simulink model "mars_rover_terrain"  (R2025a)
settings: Solver=daessc  StartTime=0.0  StopTime=130*10  FixedStep=1e-10  MaxStep=1e-1  RelTol=1e-3  AbsTol=1e-3  EnableMultiTasking=on
undefined symbols (not defined in the file): arm_q0, Control, eeConfig, L1, L2, L3, LS1, LS3, R1, R2, R3, Rover, rover_path, RS1, RS3, X, Y, Z
libraries: sm_lib x137, nesl_utility x109, fl_lib x85, sdl_lib x20, ee_lib x10, mars_rover_lib x8, simulink x4, slpidlib x3, batteryecm_lib x2, robotcorelib x1, robotalgslib x1
(part 5 of 10)

== system mars_rover_terrain/Rover/Sample/Sense Target ==
  Mux : Mux  Inputs=3
  PS-Simulink Converter : nesl_utility/PS-Simulink Converter  PhysicalDomain=network_engine_domain  SubClassName=ps_output  LeftPortType=input  RightPortType=output  PseudoPeriodic=off  Frequencies=[]  VectorFormat=1-D array  Unit=inherit  AffineConversion=off
  PS-Simulink Converter1 : nesl_utility/PS-Simulink Converter  PhysicalDomain=network_engine_domain  SubClassName=ps_output  LeftPortType=input  RightPortType=output  PseudoPeriodic=off  Frequencies=[]  VectorFormat=1-D array  Unit=inherit  AffineConversion=off
  PS-Simulink Converter2 : nesl_utility/PS-Simulink Converter  PhysicalDomain=network_engine_domain  SubClassName=ps_output  LeftPortType=input  RightPortType=output  PseudoPeriodic=off  Frequencies=[]  VectorFormat=1-D array  Unit=inherit  AffineConversion=off
  Transform Sensor : sm_lib/Frames and Transforms/Transform Sensor  MeasurementFrame=Base  RotationSequence=XYX  SenseAngle=off  SenseAxis=off  SenseQ=off  SenseR=off  SenseRotationSequence=off  SenseOmegaX=off  SenseOmegaY=off  SenseOmegaZ=off  SenseOmega=off  SenseQDot=off  SenseRDot=off  SenseRotationSequenceDot=off  SenseAlphaX=off  SenseAlphaY=off  SenseAlphaZ=off  SenseAlpha=off  SenseQDDot=off  SenseRDDot=off  SenseX=on  SenseY=on  SenseZ=on  SenseXYZ=off  SenseRad=off  SenseAzim=off  SenseDist=off  SenseInc=off  SenseXDot=off  SenseYDot=off  SenseZDot=off  SenseXYZDot=off  SenseRadDot=off  SenseAzimDot=off  SenseDistDot=off  SenseIncDot=off  SenseXDDot=off  SenseYDDot=off  SenseZDDot=off  SenseXYZDDot=off  SenseRadDDot=off  SenseAzimDDot=off  SenseDistDDot=off  SenseIncDDot=off
  ArmB : PMIOPort  Side=Right
  Target : PMIOPort  Port=2  Side=Left
  Pos : Outport
  wires:
  PS-Simulink Converter2/1 -> Mux/3
  PS-Simulink Converter1/1 -> Mux/2
  PS-Simulink Converter/1 -> Mux/1
  Mux/1 -> Pos/1  "SampleLoc"
  connections:
  PS-Simulink Converter2/LConn1 -- Transform Sensor/RConn4
  Transform Sensor/LConn1 -- ArmB/RConn1
  PS-Simulink Converter/LConn1 -- Transform Sensor/RConn2
  PS-Simulink Converter1/LConn1 -- Transform Sensor/RConn3
  Transform Sensor/RConn1 -- Target/RConn1

== system mars_rover_terrain/Rover/Sample/Subsystem ==
  In1 : Inport
  Bias : Bias  Bias=1  SaturateOnIntegerOverflow=off
  Out1 : Outport
  wires:
  Bias/1 -> Out1/1
  In1/1 -> Bias/1

== system mars_rover_terrain/Rover/Sample/Subsystem1 ==
  In1 : Inport
  Bias : Bias  Bias=1  SaturateOnIntegerOverflow=off
  m : Outport
  wires:
  In1/1 -> Bias/1
  Bias/1 -> m/1

== system mars_rover_terrain/Rover/Terrain/Contact ==
  Contact L1 : sm_lib/Forces and Torques/Spatial Contact Force  SenseSeparationDistance=off  NormalForceType=SmoothSpringDamper  NormalStiffness=contact_k  NormalStiffnessUnits=N/m  NormalDamping=contact_d  NormalDampingUnits=N/(m/s)  NormalTransitionRegionWidth=contact_tw  NormalTransitionRegionWidthUnits=m  FrictionType=SmoothStickSlip  CoefficientOfStaticFriction=friction_mus  CoefficientOfDynamicFriction=friction_mud  FrictionalCriticalVelocity=friction_vcrit  FrictionalCriticalVelocityUnits=m/s  SenseContactSignal=off  SensePenetrationDepth=off  SenseNormalVelocity=off  SenseTangentialVelocity=off  SensingForceTorqueDirection=BaseOnFollower  SensingForceTorqueResolutionFrame=ContactFrame  SenseNormalForce=off  SenseNormalForceMagnitude=off  SenseNormalTorque=off  SenseFrictionalForce=off  SenseFrictionalForceMagnitude=off  SenseFrictionalTorque=off  SenseTotalForce=off  SenseTotalTorque=off  SenseContactBaseRotation=off  SenseContactBaseTranslation=off  SenseContactFollowerRotation=off  SenseContactFollowerTranslation=off  ZeroCrossDetectContactStartAndEnd=off
  Contact L2 : sm_lib/Forces and Torques/Spatial Contact Force  SenseSeparationDistance=off  NormalForceType=SmoothSpringDamper  NormalStiffness=contact_k  NormalStiffnessUnits=N/m  NormalDamping=contact_d  NormalDampingUnits=N/(m/s)  NormalTransitionRegionWidth=contact_tw  NormalTransitionRegionWidthUnits=m  FrictionType=SmoothStickSlip  CoefficientOfStaticFriction=friction_mus  CoefficientOfDynamicFriction=friction_mud  FrictionalCriticalVelocity=friction_vcrit  FrictionalCriticalVelocityUnits=m/s  SenseContactSignal=off  SensePenetrationDepth=off  SenseNormalVelocity=off  SenseTangentialVelocity=off  SensingForceTorqueDirection=BaseOnFollower  SensingForceTorqueResolutionFrame=ContactFrame  SenseNormalForce=off  SenseNormalForceMagnitude=off  SenseNormalTorque=off  SenseFrictionalForce=off  SenseFrictionalForceMagnitude=off  SenseFrictionalTorque=off  SenseTotalForce=off  SenseTotalTorque=off  SenseContactBaseRotation=off  SenseContactBaseTranslation=off  SenseContactFollowerRotation=off  SenseContactFollowerTranslation=off  ZeroCrossDetectContactStartAndEnd=off
  Contact L3 : sm_lib/Forces and Torques/Spatial Contact Force  SenseSeparationDistance=off  NormalForceType=SmoothSpringDamper  NormalStiffness=contact_k  NormalStiffnessUnits=N/m  NormalDamping=contact_d  NormalDampingUnits=N/(m/s)  NormalTransitionRegionWidth=contact_tw  NormalTransitionRegionWidthUnits=m  FrictionType=SmoothStickSlip  CoefficientOfStaticFriction=friction_mus  CoefficientOfDynamicFriction=friction_mud  FrictionalCriticalVelocity=friction_vcrit  FrictionalCriticalVelocityUnits=m/s  SenseContactSignal=off  SensePenetrationDepth=off  SenseNormalVelocity=off  SenseTangentialVelocity=off  SensingForceTorqueDirection=BaseOnFollower  SensingForceTorqueResolutionFrame=ContactFrame  SenseNormalForce=off  SenseNormalForceMagnitude=off  SenseNormalTorque=off  SenseFrictionalForce=off  SenseFrictionalForceMagnitude=off  SenseFrictionalTorque=off  SenseTotalForce=off  SenseTotalTorque=off  SenseContactBaseRotation=off  SenseContactBaseTranslation=off  SenseContactFollowerRotation=off  SenseContactFollowerTranslation=off  ZeroCrossDetectContactStartAndEnd=off
  Contact R1 : sm_lib/Forces and Torques/Spatial Contact Force  SenseSeparationDistance=off  NormalForceType=SmoothSpringDamper  NormalStiffness=contact_k  NormalStiffnessUnits=N/m  NormalDamping=contact_d  NormalDampingUnits=N/(m/s)  NormalTransitionRegionWidth=contact_tw  NormalTransitionRegionWidthUnits=m  FrictionType=SmoothStickSlip  CoefficientOfStaticFriction=friction_mus  CoefficientOfDynamicFriction=friction_mud  FrictionalCriticalVelocity=friction_vcrit  FrictionalCriticalVelocityUnits=m/s  SenseContactSignal=off  SensePenetrationDepth=off  SenseNormalVelocity=off  SenseTangentialVelocity=off  SensingForceTorqueDirection=BaseOnFollower  SensingForceTorqueResolutionFrame=ContactFrame  SenseNormalForce=off  SenseNormalForceMagnitude=off  SenseNormalTorque=off  SenseFrictionalForce=off  SenseFrictionalForceMagnitude=off  SenseFrictionalTorque=off  SenseTotalForce=off  SenseTotalTorque=off  SenseContactBaseRotation=off  SenseContactBaseTranslation=off  SenseContactFollowerRotation=off  SenseContactFollowerTranslation=off  ZeroCrossDetectContactStartAndEnd=off
  Contact R2 : sm_lib/Forces and Torques/Spatial Contact Force  SenseSeparationDistance=off  NormalForceType=SmoothSpringDamper  NormalStiffness=contact_k  NormalStiffnessUnits=N/m  NormalDamping=contact_d  NormalDampingUnits=N/(m/s)  NormalTransitionRegionWidth=contact_tw  NormalTransitionRegionWidthUnits=m  FrictionType=SmoothStickSlip  CoefficientOfStaticFriction=friction_mus  CoefficientOfDynamicFriction=friction_mud  FrictionalCriticalVelocity=friction_vcrit  FrictionalCriticalVelocityUnits=m/s  SenseContactSignal=off  SensePenetrationDepth=off  SenseNormalVelocity=off  SenseTangentialVelocity=off  SensingForceTorqueDirection=BaseOnFollower  SensingForceTorqueResolutionFrame=ContactFrame  SenseNormalForce=off  SenseNormalForceMagnitude=off  SenseNormalTorque=off  SenseFrictionalForce=off  SenseFrictionalForceMagnitude=off  SenseFrictionalTorque=off  SenseTotalForce=off  SenseTotalTorque=off  SenseContactBaseRotation=off  SenseContactBaseTranslation=off  SenseContactFollowerRotation=off  SenseContactFollowerTranslation=off  ZeroCrossDetectContactStartAndEnd=off
  Contact R3 : sm_lib/Forces and Torques/Spatial Contact Force  SenseSeparationDistance=off  NormalForceType=SmoothSpringDamper  NormalStiffness=contact_k  NormalStiffnessUnits=N/m  NormalDamping=contact_d  NormalDampingUnits=N/(m/s)  NormalTransitionRegionWidth=contact_tw  NormalTransitionRegionWidthUnits=m  FrictionType=SmoothStickSlip  CoefficientOfStaticFriction=friction_mus  CoefficientOfDynamicFriction=friction_mud  FrictionalCriticalVelocity=friction_vcrit  FrictionalCriticalVelocityUnits=m/s  SenseContactSignal=off  SensePenetrationDepth=off  SenseNormalVelocity=off  SenseTangentialVelocity=off  SensingForceTorqueDirection=BaseOnFollower  SensingForceTorqueResolutionFrame=ContactFrame  SenseNormalForce=off  SenseNormalForceMagnitude=off  SenseNormalTorque=off  SenseFrictionalForce=off  SenseFrictionalForceMagnitude=off  SenseFrictionalTorque=off  SenseTotalForce=off  SenseTotalTorque=off  SenseContactBaseRotation=off  SenseContactBaseTranslation=off  SenseContactFollowerRotation=off  SenseContactFollowerTranslation=off  ZeroCrossDetectContactStartAndEnd=off
  Simscape Bus : SimscapeBus  HierarchyStrings=L1;L2;L3;R1;R2;R3
  Wheels : PMIOPort  Side=Right
  Surface : PMIOPort  Port=2  Side=Right
  connections:
  Contact R2/RConn1 -- Simscape Bus/LConn5
  Contact L2/RConn1 -- Simscape Bus/LConn2
  Contact L1/LConn1 -- Contact L2/LConn1 -- Contact L3/LConn1 -- Surface/RConn1 -- Contact R1/LConn1 -- Contact R3/LConn1 -- Contact R2/LConn1
  Contact L1/RConn1 -- Simscape Bus/LConn1
  Contact R3/RConn1 -- Simscape Bus/LConn6
  Simscape Bus/RConn1 -- Wheels/RConn1
  Contact R1/RConn1 -- Simscape Bus/LConn4
  Contact L3/RConn1 -- Simscape Bus/LConn3

== system mars_rover_terrain/Control/Arm Control/ Trajectory Planner/Check Drift ==
  Sensor : Inport
  IK Target : Inport  Port=2
  Demux : Demux  Outputs=3
  Demux1 : Demux  Outputs=3
  Mux : Mux  Inputs=2
  Mux1 : Mux  Inputs=2
  Mux2 : Mux  Inputs=2
  Scope1 : Scope  NumInputPorts=3
      settings: ActiveDisplayYMinimum=-0.42564  ActiveDisplayYMaximum=-0.41525  DataLoggingVariableName=ScopeData2
  wires:
  Mux2/1 -> Scope1/3
  Demux/2 -> Mux1/1
  Demux/3 -> Mux2/1
  Mux1/1 -> Scope1/2
  Demux/1 -> Mux/1
  Demux1/1 -> Mux/2
  Mux/1 -> Scope1/1
  Demux1/2 -> Mux1/2
  Demux1/3 -> Mux2/2
  IK Target/1 -> Demux1/1
  Sensor/1 -> Demux/1

== system mars_rover_terrain/Control/Arm Control/ Trajectory Planner/Planner Subsystem ==
  qJoints : Inport
  SamplePosition : Inport  Port=2
  Hold : Inport  Port=3
  Stored : Inport  Port=4
  Enable : EnablePort
  Add2 : Sum  Inputs=+-
  Clock3 : Clock
  Clock4 : Clock
  Constant2 : Constant  Value=eeConfig.Targets{:,:}
  Constant3 : Constant  Value=eeConfig.Joint_IG{:,:}
  Inverse Kinematics : MATLAB Function  TreatAsAtomicUnit=on
  Memory : Memory
  Task Scheduler : MATLAB Function  TreatAsAtomicUnit=on
  Terminator2 : Terminator
  Terminator3 : Terminator
  Transpose : Math  Operator=transpose
  Trapezoidal Velocity Profile Trajectory : robotcorelib/Trapezoidal Velocity Profile Trajectory  WaypointSource=External  Waypoints=[ 0, -0.5, -1; 0, 0.5, 1 ]  NumParams=1  Parameter1=End Time  Parameter2=End Time  ParameterSource=Internal  PeakVelocity=1  Acceleration=[ 1; 2 ]  EndTime=5  AccelTime=[ 1; 2 ]  SimulateUsing=Code generation
  Unit Delay1 : UnitDelay  InitialCondition=zeros(7,6)  SampleTime=-1  HasFrameUpgradeWarning=on
  qCmd : Outport
  CmdHold : Outport  Port=2
  CmdStored : Outport  Port=3
  Rover Mode : Outport  Port=4
  wires:
  Task Scheduler/4(sampleDropCmd) -> CmdStored/1
  SamplePosition/1 -> Inverse Kinematics/3(samplePosition)
  Task Scheduler/3(samplePickCmd) -> CmdHold/1
  qJoints/1 -> Task Scheduler/1(actJointAngles)
  Hold/1 -> Task Scheduler/3(samplePickSense)
  Stored/1 -> Task Scheduler/4(sampleDropSense)
  Trapezoidal Velocity Profile Trajectory/1 -> qCmd/1
  Constant3/1 -> Inverse Kinematics/2(eeIgs)
  Constant2/1 -> Inverse Kinematics/1(eePoseDes)
  Inverse Kinematics/1(jointSpaceWayPts) -> Unit Delay1/1, Task Scheduler/2(desJointAngles)
  Unit Delay1/1 -> Inverse Kinematics/4(prevWayPts)
  Clock3/1 -> Task Scheduler/5(currentTime)
  Clock4/1 -> Add2/1
  Trapezoidal Velocity Profile Trajectory/3 -> Terminator3/1
  Trapezoidal Velocity Profile Trajectory/2 -> Terminator2/1
  Task Scheduler/2(reset_t) -> Add2/2
  Task Scheduler/1(wayPts) -> Transpose/1
  Transpose/1 -> Trapezoidal Velocity Profile Trajectory/2
  Add2/1 -> Trapezoidal Velocity Profile Trajectory/1
  Task Scheduler/5(roverMode) -> Memory/1, Rover Mode/1
  Memory/1 -> Task Scheduler/6(roverModePrev)

== system mars_rover_terrain/Control/Arm Control/ Trajectory Planner/SampleDropOffCmdLogic ==
  u : Inport
  Constant2 : Constant
  Data Type Conversion : DataTypeConversion  OutDataTypeStr=double  SaturateOnIntegerOverflow=off  RndMeth=Floor
  Delay : Delay
  Enabled Subsystem1 : Subsystem  TreatAsAtomicUnit=on
      settings: MinAlgLoopOccurrences=on
  y : Outport
  wires:
  Delay/1 -> y/1
  Enabled Subsystem1/1(Out1) -> Delay/1
  Data Type Conversion/1 -> Enabled Subsystem1/Enable
  Constant2/1 -> Enabled Subsystem1/1(In1)
  u/1 -> Data Type Conversion/1

== system mars_rover_terrain/Control/Arm Control/ Trajectory Planner/SampleLoc wrt arm base ==
  Enable : Inport
  SampleLoc : Inport  Port=2
  Constant2 : Constant
  Enabled Subsystem1 : Subsystem  TreatAsAtomicUnit=on
      settings: MinAlgLoopOccurrences=on
  Switch : Switch  Criteria=u2 > Threshold  SaturateOnIntegerOverflow=off  InputSameDT=off
  Transpose1 : Math  Operator=transpose
  Unit Delay : UnitDelay  SampleTime=-1  HasFrameUpgradeWarning=on
  SamplePos : Outport
  wires:
  Constant2/1 -> Enabled Subsystem1/1(In1)
  SampleLoc/1 -> Switch/3
  Unit Delay/1 -> Switch/1, Transpose1/1
  Switch/1 -> Unit Delay/1
  Enable/1 -> Enabled Subsystem1/Enable
  Enabled Subsystem1/1(Out1) -> Switch/2
  Transpose1/1 -> SamplePos/1

== system mars_rover_terrain/Control/Arm Control/ Trajectory Planner/SamplePickUpCmdLogic ==
  u : Inport
  Constant2 : Constant
  Data Type Conversion : DataTypeConversion  OutDataTypeStr=double  SaturateOnIntegerOverflow=off  RndMeth=Floor
  Delay : Delay
  Enabled Subsystem1 : Subsystem  TreatAsAtomicUnit=on
      settings: MinAlgLoopOccurrences=on
  y : Outport
  wires:
  u/1 -> Data Type Conversion/1
  Constant2/1 -> Enabled Subsystem1/1(In1)
  Enabled Subsystem1/1(Out1) -> Delay/1
  Delay/1 -> y/1
  Data Type Conversion/1 -> Enabled Subsystem1/Enable

== system mars_rover_terrain/Control/Arm Control/ Trajectory Planner/hold1 ==
  Enable : Inport
  AND : Logic  IconShape=distinctive  AllPortsSameDT=off  OutDataTypeStr=boolean
  Clock : Clock
  Constant1 : Constant
  Constant3 : Constant
  Detect Rise Positive : simulink/Logic and Bit Operations/Detect Rise Positive  vinit=0  OutDataTypeStr=boolean
  Display : Display
  GreaterThanOrEqual : RelationalOperator  OutDataTypeStr=boolean  RndMeth=Simplest  InputSameDT=off
  Memory : Memory
  Switch : Switch  Criteria=u2 > Threshold  SaturateOnIntegerOverflow=off  InputSameDT=off
  plan : Outport
  wires:
  Enable/1 -> Detect Rise Positive/1
  Switch/1 -> plan/1, Display/1, Memory/1
  Constant1/1 -> Switch/1
  Clock/1 -> GreaterThanOrEqual/1
  Constant3/1 -> GreaterThanOrEqual/2
  GreaterThanOrEqual/1 -> AND/2
  AND/1 -> Switch/2
  Memory/1 -> Switch/3
  Detect Rise Positive/1 -> AND/1

== system mars_rover_terrain/Control/Arm Control/ Trajectory Planner/hold2 ==
  Enable : Inport
  AND : Logic  IconShape=distinctive  AllPortsSameDT=off  OutDataTypeStr=boolean
  Clock : Clock
  Constant1 : Constant
  Constant3 : Constant
  Detect Rise Positive : simulink/Logic and Bit Operations/Detect Rise Positive  vinit=0  OutDataTypeStr=boolean
  GreaterThanOrEqual : RelationalOperator  OutDataTypeStr=boolean  RndMeth=Simplest  InputSameDT=off
  Memory : Memory
  Switch : Switch  Criteria=u2 > Threshold  SaturateOnIntegerOverflow=off  InputSameDT=off
  plan : Outport
  wires:
  Enable/1 -> Detect Rise Positive/1
  Switch/1 -> Memory/1, plan/1
  Constant1/1 -> Switch/1
  Clock/1 -> GreaterThanOrEqual/1
  Constant3/1 -> GreaterThanOrEqual/2
  GreaterThanOrEqual/1 -> AND/2
  AND/1 -> Switch/2
  Memory/1 -> Switch/3
  Detect Rise Positive/1 -> AND/1

== system mars_rover_terrain/Control/Chassis Control/Ackerman Steer Angle/Hold Steer at Goal ==
  d : Inport
  Enable : EnablePort
  d_h : Outport
  wires:
  d/1 -> d_h/1

== system mars_rover_terrain/Control/Chassis Control/Steering Controller/Bus to Vec ==
  B : Inport
  Bus Selector : BusSelector  OutputSignals=q.L3,q.L1,q.R3,q.R1
  Mux : Mux
  V : Outport
  wires:
  Bus Selector/1 -> Mux/1  "<L3>"
  Bus Selector/4 -> Mux/4  "<R1>"
  Mux/1 -> V/1
  Bus Selector/2 -> Mux/2  "<L1>"
  Bus Selector/3 -> Mux/3  "<R3>"
  B/1 -> Bus Selector/1

== system mars_rover_terrain/Control/Chassis Control/Steering Controller/Check Difference ==
  tgt : Inport
  meas : Inport  Port=2
  Demux1 : Demux
  Demux2 : Demux
  Mux{,1..3} (4 alike) : Mux  Inputs=2
  L3 : Outport
  L1 : Outport  Port=2
  R3 : Outport  Port=3
  R1 : Outport  Port=4
  wires:
  Demux2/1 -> Mux/2
  Demux1/3 -> Mux2/1
  Demux1/2 -> Mux1/1
  Demux2/4 -> Mux3/2
  Demux2/2 -> Mux1/2
  Demux2/3 -> Mux2/2
  meas/1 -> Demux2/1
  Demux1/1 -> Mux/1
  Mux1/1 -> L1/1
  Demux1/4 -> Mux3/1
  Mux3/1 -> R1/1
  Mux2/1 -> R3/1
  Mux/1 -> L3/1
  tgt/1 -> Demux1/1

== system mars_rover_terrain/Control/Chassis Control/Steering Controller/Filter qMeas ==
  In : Inport
  Gain : Gain  Gain=1./b
  Integrator : Integrator  InitialCondition=x_initial.*b
  Sum : Sum  Inputs=|+-  InputSameDT=on  SaturateOnIntegerOverflow=on  OutDataTypeStr=Inherit: Same as first input
  Out : Outport  VectorParamsAs1DForOutWhenUnconnected=off
  wires:
  Sum/1 -> Integrator/1
  In/1 -> Sum/1
  Integrator/1 -> Gain/1
  Gain/1 -> Sum/2, Out/1

== system mars_rover_terrain/Control/Chassis Control/Steering Controller/Filter qTarget ==
  In : Inport
  Gain : Gain  Gain=1./b
  Integrator : Integrator  InitialCondition=x_initial.*b
  Sum : Sum  Inputs=|+-  InputSameDT=on  SaturateOnIntegerOverflow=on  OutDataTypeStr=Inherit: Same as first input
  Out : Outport  VectorParamsAs1DForOutWhenUnconnected=off
  wires:
  Gain/1 -> Out/1, Sum/2
  Integrator/1 -> Gain/1
  In/1 -> Sum/1
  Sum/1 -> Integrator/1

== system mars_rover_terrain/Control/Chassis Control/Target Direction and Speed/Check Distance To Goal ==
  note: Distance from Goal to satisfy that the robot has reached the goal
  goal : Inport
  currentPose : Inport  Port=2
  linVel : Inport  Port=3
  Add : Sum
  Constant : Constant  Value=0.25
  Constant1 : Constant  Value=2*Control.Drive.TargetAccel
  Divide : Product  Inputs=*/
  Dot Product : DotProduct  OutDataTypeStr=Inherit: Inherit via internal rule
  Gain1 : Gain
  Less Than : RelationalOperator  Operator=>  OutDataTypeStr=boolean  RndMeth=Simplest  InputSameDT=off
  Less Than1 : RelationalOperator  Operator=>  OutDataTypeStr=boolean  RndMeth=Simplest  InputSameDT=off
  NOT : Logic  Operator=NOT  IconShape=distinctive  AllPortsSameDT=off  OutDataTypeStr=boolean
  Scope1 : Scope
      settings: ActiveDisplayYMinimum=-1.62385  ActiveDisplayYMaximum=15.54178  DataLoggingVariableName=ScopeData17
  Selector : Selector  InputPortWidth=3  IndexOptions=Index vector (dialog)  Indices=[1 2]  OutputSizes=1
  Sqrt : Sqrt
  Subtract : Sum  Inputs=+-
  Unit Delay : UnitDelay  SampleTime=-1  HasFrameUpgradeWarning=on
  const : Math  Operator=square
  atGoal : Outport
  Slow : Outport  Port=2
  wires:
  goal/1 -> Subtract/2
  Dot Product/1 -> Sqrt/1
  Constant/1 -> Gain1/1, Less Than/2
  currentPose/1 -> Selector/1
  Sqrt/1 -> Scope1/1, Less Than/1, Less Than1/1
  Subtract/1 -> Dot Product/2, Dot Product/1
  Selector/1 -> Subtract/1
  linVel/1 -> const/1
  const/1 -> Divide/1
  Constant1/1 -> Divide/2
  Less Than1/1 -> Slow/1
  Add/1 -> Less Than1/2
  Divide/1 -> Add/1
  Gain1/1 -> Add/2
  Less Than/1 -> NOT/1
  NOT/1 -> Unit Delay/1
  Unit Delay/1 -> atGoal/1

== system mars_rover_terrain/Control/Chassis Control/Target Direction and Speed/hold ==
  In1 : Inport
  Constant9 : Constant  Value=inf
  NOT1 : Logic  Operator=NOT  IconShape=distinctive  AllPortsSameDT=off  OutDataTypeStr=boolean
  RoverStopTime : Subsystem
  Switch3 : Switch  Criteria=u2 > Threshold  SaturateOnIntegerOverflow=off  InputSameDT=off
  Unit Delay1 : UnitDelay  SampleTime=-1  HasFrameUpgradeWarning=on
  Out1 : Outport
  wires:
  Unit Delay1/1 -> Switch3/2
  RoverStopTime/1(DeAccelTime) -> Switch3/1
  Switch3/1 -> Out1/1
  NOT1/1 -> RoverStopTime/1(Enable), Unit Delay1/1
  Constant9/1 -> Switch3/3
  In1/1 -> NOT1/1

== system mars_rover_terrain/Control/Chassis Control/Wheel Speed Controller/Bus to Vec ==
  B : Inport
  Bus Selector : BusSelector  OutputSignals=w.L1,w.L2,w.L3,w.R1,w.R2,w.R3
  Mux : Mux  Inputs=6
  V : Outport
  wires:
  Bus Selector/1 -> Mux/1  "<L1>"
  Bus Selector/3 -> Mux/3  "<L3>"
  Bus Selector/4 -> Mux/4  "<R1>"
  Bus Selector/6 -> Mux/6  "<R3>"
  Bus Selector/5 -> Mux/5  "<R2>"
  Bus Selector/2 -> Mux/2  "<L2>"
  B/1 -> Bus Selector/1
  Mux/1 -> V/1

== system mars_rover_terrain/Control/Chassis Control/Wheel Speed Controller/Filter wMeas ==
  In : Inport
  Gain : Gain  Gain=1./b
  Integrator : Integrator  InitialCondition=x_initial.*b
  Sum : Sum  Inputs=|+-  InputSameDT=on  SaturateOnIntegerOverflow=on  OutDataTypeStr=Inherit: Same as first input
  Out : Outport  VectorParamsAs1DForOutWhenUnconnected=off
  wires:
  Sum/1 -> Integrator/1
  In/1 -> Sum/1
  Integrator/1 -> Gain/1
  Gain/1 -> Sum/2, Out/1

== system mars_rover_terrain/Control/Chassis Control/Wheel Speed Controller/Filter wTarget ==
  In : Inport
  Gain : Gain  Gain=1./b
  Integrator : Integrator  InitialCondition=x_initial.*b
  Sum : Sum  Inputs=|+-  InputSameDT=on  SaturateOnIntegerOverflow=on  OutDataTypeStr=Inherit: Same as first input
  Out : Outport  VectorParamsAs1DForOutWhenUnconnected=off
  wires:
  Gain/1 -> Out/1, Sum/2
  Integrator/1 -> Gain/1
  In/1 -> Sum/1
  Sum/1 -> Integrator/1

== system mars_rover_terrain/Rover/Chassis/Camera/rsm_base_1_RIGID ==
  ReferenceFrame : sm_lib/Frames and Transforms/Reference Frame
  Solid : sm_lib/Body Elements/File Solid  ExtGeomFileName=rover_chassis_sensor_base.stl  UnitType=Custom  ExtGeomFileUnits=cm  StepReaderType=HEX  ExportConvexHullGeometry=off  InertiaType=CalculateFromGeometry  BasedOnType=Density  Density=2000  DensityUnits=kg/m^3  Mass=202690.508551217  MassUnits=kg  CenterOfMass=[-2.09994238818055e-07 21.8231915316941 -2.20167989735098e-07]  CenterOfMassUnits=m  MomentsOfInertia=[2411866.97125594 5940029.20050206 6701187.74240286]  MomentsOfInertiaUnits=kg*m^2  ProductsOfInertia=[0.00792234309140369 -0.0164088810985133 -0.460936358460458]  ProductsOfInertiaUnits=kg*m^2  GraphicType=FromGeometry  MarkerShape=Sphere  MarkerSize=10  GraphicVisPropType=SimpleVisualProperties  GraphicDiffuseColor=[0.2 0.2 0.2]  GraphicOpacity=1  GraphicSpecularColor=[0.5 0.5 0.5 1.0]  GraphicAmbientColor=[0.15 0.15 0.15 1.0]  GraphicEmissiveColor=[0.0 0.0 0.0 1.0]  GraphicShininess=75  DoExposeReferenceFrame=on  SerializedFrames=<Frames/>
  Transform : sm_lib/Frames and Transforms/Rigid Transform  RotationMethod=ArbitraryAxis  FollAlignAxisA=+X  BaseAlignAxisA=+Y  FollAlignAxisB=+Y  BaseAlignAxisB=+Z  RotationStandardAxis=+Z  RotationAngle=2.0943951023932  RotationAngleUnits=rad  RotationArbitraryAxis=[0.577350269189626 0.577350269189626 0.577350269189626]  RotationSequenceAxes=FollowerAxes  RotationSequence=XYX  RotationSequenceAngles=[0 0 0]  RotationSequenceAnglesUnits=deg  RotationMatrix=[1 0 0; 0 1 0; 0 0 1]  Quaternion=[1 0 0 0]  TranslationMethod=Cartesian  TranslationCartesianOffset=[-40 220.000003786473 -2.05636384635e-06]  TranslationCartesianOffsetUnits=mm  TranslationStandardAxis=+Z  TranslationStandardOffset=0  TranslationStandardOffsetUnits=mm  TranslationROffset=0  TranslationROffsetUnits=m  TranslationThetaOffset=0  TranslationThetaOffsetUnits=deg  TranslationZOffset=0  TranslationZOffsetUnits=m
  F : PMIOPort  Side=Right
  F1 : PMIOPort  Port=2  Side=Left
  connections:
  Transform/LConn1 -- F1/RConn1 -- ReferenceFrame/RConn1 -- Solid/RConn1
  Transform/RConn1 -- F/RConn1

== system mars_rover_terrain/Rover/Chassis/Camera/rsm_head_1_RIGID ==
  Reference Camera : sm_lib/Frames and Transforms/Reference Frame
  ReferenceFrame : sm_lib/Frames and Transforms/Reference Frame
  Rigid Transform : sm_lib/Frames and Transforms/Rigid Transform  RotationMethod=StandardAxis  FollAlignAxisA=+X  BaseAlignAxisA=+Y  FollAlignAxisB=+Y  BaseAlignAxisB=+Z  RotationStandardAxis=+X  RotationAngle=-90  RotationAngleUnits=deg  RotationArbitraryAxis=[0 0 1]  RotationSequenceAxes=FollowerAxes  RotationSequence=XYX  RotationSequenceAngles=[0 0 0]  RotationSequenceAnglesUnits=deg  RotationMatrix=[1 0 0; 0 1 0; 0 0 1]  Quaternion=[1 0 0 0]  TranslationMethod=Cartesian  TranslationCartesianOffset=[12 11 13]  TranslationCartesianOffsetUnits=cm  TranslationStandardAxis=+Z  TranslationStandardOffset=0  TranslationStandardOffsetUnits=cm  TranslationROffset=0  TranslationROffsetUnits=m  TranslationThetaOffset=0  TranslationThetaOffsetUnits=deg  TranslationZOffset=0  TranslationZOffsetUnits=m
  Solid : sm_lib/Body Elements/File Solid  ExtGeomFileName=rover_chassis_sensor_head.stl  UnitType=Custom  ExtGeomFileUnits=cm  StepReaderType=HEX  ExportConvexHullGeometry=off  InertiaType=CalculateFromGeometry  BasedOnType=Density  Density=2000  DensityUnits=kg/m^3  Mass=1  MassUnits=kg  CenterOfMass=[-0.00288550161429388 71.0000014663329 -4.54954138701768e-07]  CenterOfMassUnits=m  MomentsOfInertia=[1608495.92335293 6519098.97331966 6519098.97331985]  MomentsOfInertiaUnits=kg*m^2  ProductsOfInertia=[-6.49609544482223e-08 0.336731288221059 1.08955853960892]  ProductsOfInertiaUnits=kg*m^2  GraphicType=FromGeometry  MarkerShape=Sphere  MarkerSize=10  GraphicVisPropType=SimpleVisualProperties  GraphicDiffuseColor=[0.80784315 0.80784315 0.6431373]  GraphicOpacity=1  GraphicSpecularColor=[1 1 1 1.0]  GraphicAmbientColor=[0.15 0.15 0.15 0.8]  GraphicEmissiveColor=[0 0 0 1]  GraphicShininess=90  DoExposeReferenceFrame=on  SerializedFrames=<Frames/>
  Transform : sm_lib/Frames and Transforms/Rigid Transform  RotationMethod=ArbitraryAxis  FollAlignAxisA=+X  BaseAlignAxisA=+Y  FollAlignAxisB=+Y  BaseAlignAxisB=+Z  RotationStandardAxis=+Z  RotationAngle=2.0943951023932  RotationAngleUnits=rad  RotationArbitraryAxis=[0.577350269189626 0.577350269189626 0.577350269189626]  RotationSequenceAxes=FollowerAxes  RotationSequence=XYX  RotationSequenceAngles=[0 0 0]  RotationSequenceAnglesUnits=deg  RotationMatrix=[1 0 0; 0 1 0; 0 0 1]  Quaternion=[1 0 0 0]  TranslationMethod=Cartesian  TranslationCartesianOffset=[-40.5288600921631 710.000004438766 -7.70947271803379e-06]  TranslationCartesianOffsetUnits=mm  TranslationStandardAxis=+Z  TranslationStandardOffset=0  TranslationStandardOffsetUnits=mm  TranslationROffset=0  TranslationROffsetUnits=m  TranslationThetaOffset=0  TranslationThetaOffsetUnits=deg  TranslationZOffset=0  TranslationZOffsetUnits=m
  F : PMIOPort  Side=Left
  connections:
  ReferenceFrame/RConn1 -- Solid/RConn1 -- Transform/LConn1
  Transform/RConn1 -- F/RConn1 -- Rigid Transform/LConn1
  Rigid Transform/RConn1 -- Reference Camera/RConn1

== system mars_rover_terrain/Rover/Chassis/Camera/rsm_lower_mast_2_RIGID ==
  ReferenceFrame : sm_lib/Frames and Transforms/Reference Frame
  Solid : sm_lib/Body Elements/File Solid  ExtGeomFileName=rover_chassis_sensor_mast_lower.stl  UnitType=Custom  ExtGeomFileUnits=cm  StepReaderType=HEX  ExportConvexHullGeometry=off  InertiaType=CalculateFromGeometry  BasedOnType=Density  Density=2000  DensityUnits=kg/m^3  Mass=403410.668072862  MassUnits=kg  CenterOfMass=[4.00000000041938 10.1119460218271 35.0000011171366]  CenterOfMassUnits=m  MomentsOfInertia=[4810006.95412572 3779509.77447628 5346172.06825756]  MomentsOfInertiaUnits=kg*m^2  ProductsOfInertia=[0.0256104910578052 9.59441184474277e-11 -0.00591852250388119]  ProductsOfInertiaUnits=kg*m^2  GraphicType=FromGeometry  MarkerShape=Sphere  MarkerSize=10  GraphicVisPropType=SimpleVisualProperties  GraphicDiffuseColor=[1 1 0.8]  GraphicOpacity=1  GraphicSpecularColor=[0.5 0.5 0.5 1.0]  GraphicAmbientColor=[0.15 0.15 0.15 1.0]  GraphicEmissiveColor=[0.0 0.0 0.0 1.0]  GraphicShininess=75  DoExposeReferenceFrame=on  SerializedFrames=<Frames/>
  Transform : sm_lib/Frames and Transforms/Rigid Transform  RotationMethod=ArbitraryAxis  FollAlignAxisA=+X  BaseAlignAxisA=+Y  FollAlignAxisB=+Y  BaseAlignAxisB=+Z  RotationStandardAxis=+Z  RotationAngle=2.0943951023932  RotationAngleUnits=rad  RotationArbitraryAxis=[-0.577350269189626 -0.577350269189626 -0.577350269189626]  RotationSequenceAxes=FollowerAxes  RotationSequence=XYX  RotationSequenceAngles=[0 0 0]  RotationSequenceAnglesUnits=deg  RotationMatrix=[1 0 0; 0 1 0; 0 0 1]  Quaternion=[1 0 0 0]  TranslationMethod=Cartesian  TranslationCartesianOffset=[40.0000013147577 450.900022888183 350.000005500325]  TranslationCartesianOffsetUnits=mm  TranslationStandardAxis=+Z  TranslationStandardOffset=0  TranslationStandardOffsetUnits=mm  TranslationROffset=0  TranslationROffsetUnits=m  TranslationThetaOffset=0  TranslationThetaOffsetUnits=deg  TranslationZOffset=0  TranslationZOffsetUnits=m
  Transform1 : sm_lib/Frames and Transforms/Rigid Transform  RotationMethod=ArbitraryAxis  FollAlignAxisA=+X  BaseAlignAxisA=+Y  FollAlignAxisB=+Y  BaseAlignAxisB=+Z  RotationStandardAxis=+Z  RotationAngle=2.0943951023932  RotationAngleUnits=rad  RotationArbitraryAxis=[0.577350269189626 0.577350269189626 0.577350269189626]  RotationSequenceAxes=FollowerAxes  RotationSequence=XYX  RotationSequenceAngles=[0 0 0]  RotationSequenceAnglesUnits=deg  RotationMatrix=[1 0 0; 0 1 0; 0 0 1]  Quaternion=[1 0 0 0]  TranslationMethod=Cartesian  TranslationCartesianOffset=[0 100.000002423247 350.000011189513]  TranslationCartesianOffsetUnits=mm  TranslationStandardAxis=+Z  TranslationStandardOffset=0  TranslationStandardOffsetUnits=mm  TranslationROffset=0  TranslationROffsetUnits=m  TranslationThetaOffset=0  TranslationThetaOffsetUnits=deg  TranslationZOffset=0  TranslationZOffsetUnits=m
  F1 : PMIOPort  Side=Left
  F : PMIOPort  Port=2  Side=Right
  connections:
  Transform/LConn1 -- Transform1/LConn1 -- ReferenceFrame/RConn1 -- Solid/RConn1
  Transform/RConn1 -- F/RConn1
  Transform1/RConn1 -- F1/RConn1

== system mars_rover_terrain/Rover/Chassis/Camera/rsm_outer_ring_1_RIGID ==
  ReferenceFrame : sm_lib/Frames and Transforms/Reference Frame
  Rigid Transform : sm_lib/Frames and Transforms/Rigid Transform  RotationMethod=StandardAxis  FollAlignAxisA=+X  BaseAlignAxisA=+Y  FollAlignAxisB=+Y  BaseAlignAxisB=+Z  RotationStandardAxis=+Z  RotationAngle=20.0  RotationAngleUnits=deg  RotationArbitraryAxis=[0 0 1]  RotationSequenceAxes=FollowerAxes  RotationSequence=XYX  RotationSequenceAngles=[0 0 0]  RotationSequenceAnglesUnits=deg  RotationMatrix=[1 0 0; 0 1 0; 0 0 1]  Quaternion=[1 0 0 0]  TranslationMethod=None  TranslationCartesianOffset=[0 0 0]  TranslationCartesianOffsetUnits=m  TranslationStandardAxis=+Z  TranslationStandardOffset=0  TranslationStandardOffsetUnits=m  TranslationROffset=0  TranslationROffsetUnits=m  TranslationThetaOffset=0  TranslationThetaOffsetUnits=deg  TranslationZOffset=0  TranslationZOffsetUnits=m
  Solid : sm_lib/Body Elements/File Solid  ExtGeomFileName=rover_chassis_sensor_ring_outer.stl  UnitType=Custom  ExtGeomFileUnits=cm  StepReaderType=HEX  ExportConvexHullGeometry=off  InertiaType=CalculateFromGeometry  BasedOnType=Density  Density=2000  DensityUnits=kg/m^3  Mass=2000  MassUnits=kg  CenterOfMass=[3.99999986837507 43.0793255522792 35.0000003648552]  CenterOfMassUnits=m  MomentsOfInertia=[35996.0863503472 57529.9697773705 35996.0863503472]  MomentsOfInertiaUnits=kg*m^2  ProductsOfInertia=[0.000493832044278217 -4.64395705120422e-11 0.00068000513182705]  ProductsOfInertiaUnits=kg*m^2  GraphicType=FromGeometry  MarkerShape=Sphere  MarkerSize=10  GraphicVisPropType=SimpleVisualProperties  GraphicDiffuseColor=[0.2 0.2 0.2]  GraphicOpacity=1  GraphicSpecularColor=[0.5 0.5 0.5 1.0]  GraphicAmbientColor=[0.15 0.15 0.15 1.0]  GraphicEmissiveColor=[0.0 0.0 0.0 1.0]  GraphicShininess=75  DoExposeReferenceFrame=on  SerializedFrames=<Frames/>
  Transform : sm_lib/Frames and Transforms/Rigid Transform  RotationMethod=ArbitraryAxis  FollAlignAxisA=+X  BaseAlignAxisA=+Y  FollAlignAxisB=+Y  BaseAlignAxisB=+Z  RotationStandardAxis=+Z  RotationAngle=2.09439510239319  RotationAngleUnits=rad  RotationArbitraryAxis=[-0.577350269189626 -0.577350269189627 -0.577350269189625]  RotationSequenceAxes=FollowerAxes  RotationSequence=XYX  RotationSequenceAngles=[0 0 0]  RotationSequenceAnglesUnits=deg  RotationMatrix=[1 0 0; 0 1 0; 0 0 1]  Quaternion=[1 0 0 0]  TranslationMethod=Cartesian  TranslationCartesianOffset=[39.9999957537947 420.900022888184 350.000001520764]  TranslationCartesianOffsetUnits=mm  TranslationStandardAxis=+Z  TranslationStandardOffset=0  TranslationStandardOffsetUnits=mm  TranslationROffset=0  TranslationROffsetUnits=m  TranslationThetaOffset=0  TranslationThetaOffsetUnits=deg  TranslationZOffset=0  TranslationZOffsetUnits=m
  Transform1 : sm_lib/Frames and Transforms/Rigid Transform  RotationMethod=ArbitraryAxis  FollAlignAxisA=+X  BaseAlignAxisA=+Y  FollAlignAxisB=+Y  BaseAlignAxisB=+Z  RotationStandardAxis=+Z  RotationAngle=2.29441736937637  RotationAngleUnits=rad  RotationArbitraryAxis=[-0.450882585021863 -0.631151683244211 -0.631151683244211]  RotationSequenceAxes=FollowerAxes  RotationSequence=XYX  RotationSequenceAngles=[0 0 0]  RotationSequenceAnglesUnits=deg  RotationMatrix=[1 0 0; 0 1 0; 0 0 1]  Quaternion=[1 0 0 0]  TranslationMethod=Cartesian  TranslationCartesianOffset=[39.9999957537972 461.900007629394 350.000001520762]  TranslationCartesianOffsetUnits=mm  TranslationStandardAxis=+Z  TranslationStandardOffset=0  TranslationStandardOffsetUnits=mm  TranslationROffset=0  TranslationROffsetUnits=m  TranslationThetaOffset=0  TranslationThetaOffsetUnits=deg  TranslationZOffset=0  TranslationZOffsetUnits=m
  F1 : PMIOPort  Side=Left
  F : PMIOPort  Port=2  Side=Left
  connections:
  Transform/LConn1 -- Transform1/LConn1 -- ReferenceFrame/RConn1 -- Solid/RConn1
  Transform/RConn1 -- F/RConn1
  Rigid Transform/RConn1 -- F1/RConn1
  Rigid Transform/LConn1 -- Transform1/RConn1

== system mars_rover_terrain/Rover/Chassis/Camera/rsm_upper_mast_1_RIGID ==
  ReferenceFrame : sm_lib/Frames and Transforms/Reference Frame
  Solid : sm_lib/Body Elements/File Solid  ExtGeomFileName=rover_chassis_sensor_mast_upper.stl  UnitType=Custom  ExtGeomFileUnits=cm  StepReaderType=HEX  ExportConvexHullGeometry=off  InertiaType=CalculateFromGeometry  BasedOnType=Density  Density=2000  DensityUnits=kg/m^3  Mass=382776.497765057  MassUnits=kg  CenterOfMass=[3.99998590581562 58.9787952931336 34.9999786232352]  CenterOfMassUnits=m  MomentsOfInertia=[3038949.11550358 3496444.12832479 3624138.33109519]  MomentsOfInertiaUnits=kg*m^2  ProductsOfInertia=[-149.383305940768 -0.0992863146641867 -86.2313374210248]  ProductsOfInertiaUnits=kg*m^2  GraphicType=FromGeometry  MarkerShape=Sphere  MarkerSize=10  GraphicVisPropType=SimpleVisualProperties  GraphicDiffuseColor=[1 1 0.8]  GraphicOpacity=1  GraphicSpecularColor=[0.5 0.5 0.5 1.0]  GraphicAmbientColor=[0.15 0.15 0.15 1.0]  GraphicEmissiveColor=[0.0 0.0 0.0 1.0]  GraphicShininess=75  DoExposeReferenceFrame=on  SerializedFrames=<Frames/>
  Transform : sm_lib/Frames and Transforms/Rigid Transform  RotationMethod=ArbitraryAxis  FollAlignAxisA=+X  BaseAlignAxisA=+Y  FollAlignAxisB=+Y  BaseAlignAxisB=+Z  RotationStandardAxis=+Z  RotationAngle=2.0943951023932  RotationAngleUnits=rad  RotationArbitraryAxis=[-0.577350269189626 -0.577350269189626 -0.577350269189626]  RotationSequenceAxes=FollowerAxes  RotationSequence=XYX  RotationSequenceAngles=[0 0 0]  RotationSequenceAnglesUnits=deg  RotationMatrix=[1 0 0; 0 1 0; 0 0 1]  Quaternion=[1 0 0 0]  TranslationMethod=Cartesian  TranslationCartesianOffset=[39.8936241533249 429.9 349.815749642353]  TranslationCartesianOffsetUnits=mm  TranslationStandardAxis=+Z  TranslationStandardOffset=0  TranslationStandardOffsetUnits=mm  TranslationROffset=0  TranslationROffsetUnits=m  TranslationThetaOffset=0  TranslationThetaOffsetUnits=deg  TranslationZOffset=0  TranslationZOffsetUnits=m
  Transform1 : sm_lib/Frames and Transforms/Rigid Transform  RotationMethod=ArbitraryAxis  FollAlignAxisA=+X  BaseAlignAxisA=+Y  FollAlignAxisB=+Y  BaseAlignAxisB=+Z  RotationStandardAxis=+Z  RotationAngle=2.0943951023932  RotationAngleUnits=rad  RotationArbitraryAxis=[0.577350269189626 0.577350269189626 0.577350269189626]  RotationSequenceAxes=FollowerAxes  RotationSequence=XYX  RotationSequenceAngles=[0 0 0]  RotationSequenceAnglesUnits=deg  RotationMatrix=[1 0 0; 0 1 0; 0 0 1]  Quaternion=[1 0 0 0]  TranslationMethod=Cartesian  TranslationCartesianOffset=[7.105427357601e-14 590.000009936775 350.000030393688]  TranslationCartesianOffsetUnits=mm  TranslationStandardAxis=+Z  TranslationStandardOffset=0  TranslationStandardOffsetUnits=mm  TranslationROffset=0  TranslationROffsetUnits=m  TranslationThetaOffset=0  TranslationThetaOffsetUnits=deg  TranslationZOffset=0  TranslationZOffsetUnits=m
  F : PMIOPort  Side=Left
  F1 : PMIOPort  Port=2  Side=Right
  connections:
  Transform/LConn1 -- Transform1/LConn1 -- ReferenceFrame/RConn1 -- Solid/RConn1
  Transform/RConn1 -- F/RConn1
  Transform1/RConn1 -- F1/RConn1

== system mars_rover_terrain/Rover/Chassis/Powertrain/Electrical ==
  In Bus Element : Inport  PortName=Trq  Element=Steer
  In Bus Element1 : Inport  PortName=Trq  Element=Drive
  Drive : Subsystem  mask{trq_max=Rover.Powertrain.Drive.Motor.max_torque, power_max=Rover.Powertrain.Drive.Motor.max_power, trq_tc=Rover.Powertrain.Drive.Motor.tc_torque, eff_overall=Rover.Powertrain.Drive.Motor.efficiency, eff_spd=Rover.Powertrain.Drive.Motor.eff_meas_spd, eff_trq=Rover.Powertrain.Drive.Motor.eff_meas_trq, rotor_d=Rover.Powertrain.Drive.Motor.damping, drive_ratio=Rover.Powertrain.Drive.Motor.gear_ratio}
      mask prompts: trq_max "Max Torque (N*m)"; power_max "Max Power (W)"; trq_tc "Time Constant, Torque (s)"; eff_overall "Efficiency (%)"; eff_spd "Speed for Efficiency (rpm)"; eff_trq "Torque for Efficiency (N*m)"; rotor_d "Rotor Damping (N*m/(rad/s))"; drive_ratio "Drive Ratio"
      mask Display: image('mars_rover_terrain_motor_elec_drive.png');
  Mechanical Rotational Reference : fl_lib/Mechanical/Rotational Elements/Mechanical Rotational Reference
  Power : Subsystem
      mask Display: image('mars_rover_terrain_battery.png');
  Steer : Subsystem  mask{trq_max=Rover.Powertrain.Steer.Motor.max_torque, power_max=Rover.Powertrain.Steer.Motor.max_power, trq_tc=Rover.Powertrain.Steer.Motor.tc_torque, eff_overall=Rover.Powertrain.Steer.Motor.efficiency, eff_spd=Rover.Powertrain.Steer.Motor.eff_meas_spd, eff_trq=Rover.Powertrain.Steer.Motor.eff_meas_trq, rotor_d=Rover.Powertrain.Steer.Motor.damping, drive_ratio=Rover.Powertrain.Steer.Motor.gear_ratio}
      mask prompts: trq_max "Max Torque (N*m)"; power_max "Max Power (W)"; trq_tc "Time Constant, Torque (s)"; eff_overall "Efficiency (%)"; eff_spd "Speed for Efficiency (rpm)"; eff_trq "Torque for Efficiency (N*m)"; rotor_d "Rotor Damping (N*m/(rad/s))"; drive_ratio "Drive Ratio"
      mask Display: image('mars_rover_terrain_motor_elec_steer.png');
  S : PMIOPort  Side=Right
  Out Bus Element : Outport  PortName=m  Element=Drive
  Out Bus Element1 : Outport  PortName=m  Element=Steer
  Out Bus Element2 : Outport  PortName=m  Element=Battery
  wires:
  In Bus Element/1 -> Steer/1(Trq)
  In Bus Element1/1 -> Drive/1(Trq)
  Steer/1(m) -> Out Bus Element1/1
  Drive/1(m) -> Out Bus Element/1
  Power/1(m) -> Out Bus Element2/1
  connections:
  S/RConn1 -- Drive/RConn1 -- Steer/RConn1
  Power/RConn1 -- Drive/LConn1 -- Steer/LConn1
  Mechanical Rotational Reference/LConn1 -- Drive/RConn2 -- Steer/RConn2
  Power/RConn2 -- Drive/LConn2 -- Steer/LConn2

== system mars_rover_terrain/Rover/Chassis/Powertrain/Ideal ==
  In Bus Element6 : Inport  PortName=Trq  Element=Steer
  In Bus Element : Inport  PortName=Trq  Element=Drive
  Calculate Power : Subsystem
  Drive : Subsystem  mask{drive_ratio=Rover.Powertrain.Drive.Motor.gear_ratio, motor_d=Rover.Powertrain.Drive.Motor.damping, motor_tc=Rover.Powertrain.Drive.Motor.tc_torque}
      mask prompts: drive_ratio "Drive Ratio"; motor_d "Motor Damping (N*m/(rad/s))"; motor_tc "Motor Time Constant"
      mask Display: image('mars_rover_terrain_motor_ideal_drive.png');
  Mechanical Rotational Reference : fl_lib/Mechanical/Rotational Elements/Mechanical Rotational Reference
  Power : Subsystem
      mask Display: image('mars_rover_terrain_battery.png');
  Steer : Subsystem  mask{drive_ratio=Rover.Powertrain.Drive.Motor.gear_ratio, motor_d=Rover.Powertrain.Steer.Motor.damping, motor_tc=Rover.Powertrain.Steer.Motor.tc_torque}
      mask prompts: drive_ratio "Gear Ratio"; motor_d "Motor Damping (N*m/(rad/s))"; motor_tc "Motor Time Constant"
      mask Display: image('mars_rover_terrain_motor_ideal_steer.png')
  S : PMIOPort  Side=Right
  Out Bus Element : Outport  PortName=m  Element=Steer
  Out Bus Element1 : Outport  PortName=m  Element=Drive
  Out Bus Element2 : Outport  PortName=m  Element=Battery
  wires:
  Steer/1(m) -> Out Bus Element/1, [S]
  In Bus Element6/1 -> Steer/1(Trq)
  Drive/1(m) -> [D], Out Bus Element1/1
  In Bus Element/1 -> Drive/1(Trq)
  [S] -> Calculate Power/1(S)
  [D] -> Calculate Power/2(D)
  Calculate Power/1(i) -> Power/1(i)
  Power/1(m) -> Out Bus Element2/1
  connections:
  Steer/RConn1 -- Drive/RConn1 -- S/RConn1
  Mechanical Rotational Reference/LConn1 -- Steer/LConn1 -- Drive/LConn1
